simulink model "Woofer_Vented_L160_simscape"  (R2026a)
settings: Solver=ode23t  StopTime=0.2
libraries: fl_lib x21, nesl_utility x6
settings Model: Creator=mads  LastModifiedBy=mads
settings DataIOCC: ExternalInput=[(0:1e-4:0.2)' sin(2*pi*25*(0:1e-4:0.2)')]  LoadExternalInput=on

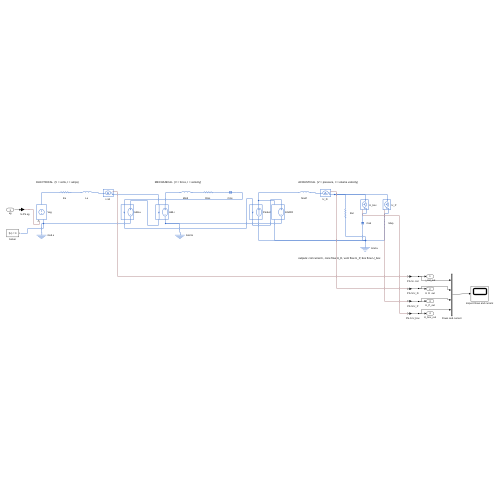
[thumbnail: Simulink's stored preview of the top-level diagram]
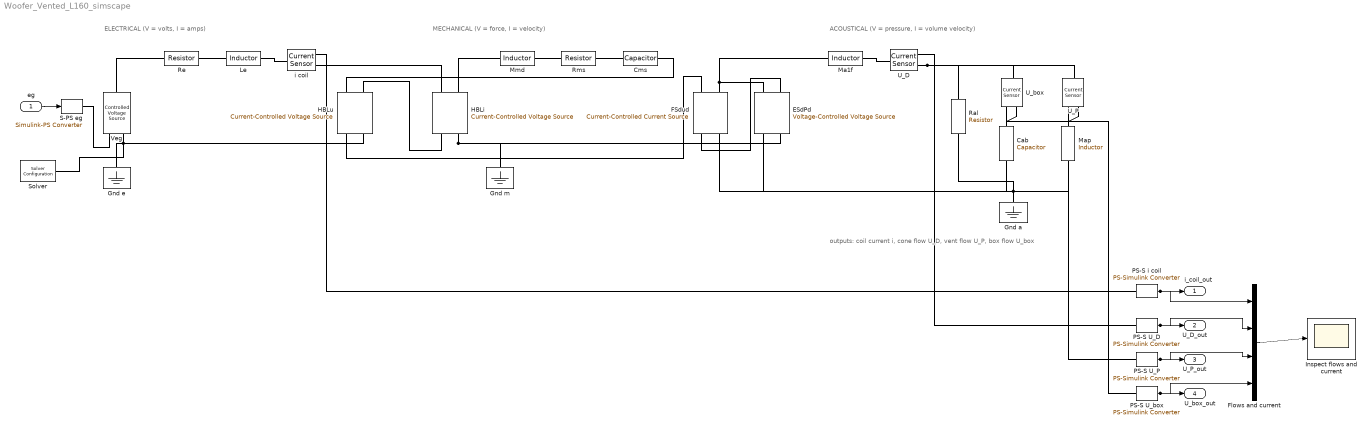
== system Woofer_Vented_L160_simscape ==
  note: ELECTRICAL (V = volts, I = amps)
  note: MECHANICAL (V = force, I = velocity)
  note: ACOUSTICAL (V = pressure, I = volume velocity)
  note: outputs: coil current i, cone flow U_D, vent flow U_P, box flow U_box
  eg : Inport
  Cab : fl_lib/Electrical/Electrical Elements/Capacitor  c=6.21e-07 F  r=0 Ohm  g=0 1/Ohm  i_specify=off  i_priority=None  i=0 A  i_nominal_specify=off  i_nominal_value=1  i_nominal_unit=A  v_specify=off  v_priority=None  v=0 V  v_nominal_specify=off  v_nominal_value=1  v_nominal_unit=V  vc_specify=off  vc_priority=High  vc=0 V  vc_nominal_specify=off  vc_nominal_value=1  vc_nominal_unit=V
  Cms : fl_lib/Electrical/Electrical Elements/Capacitor  c=0.0011735 F  r=0 Ohm  g=0 1/Ohm  i_specify=off  i_priority=None  i=0 A  i_nominal_specify=off  i_nominal_value=1  i_nominal_unit=A  v_specify=off  v_priority=None  v=0 V  v_nominal_specify=off  v_nominal_value=1  v_nominal_unit=V  vc_specify=off  vc_priority=High  vc=0 V  vc_nominal_specify=off  vc_nominal_value=1  vc_nominal_unit=V
  ESdPd : fl_lib/Electrical/Electrical Sources/Voltage-Controlled Voltage Source  K=0.034967  v1_specify=off  v1_priority=None  v1=0 V  v1_nominal_specify=off  v1_nominal_value=1  v1_nominal_unit=V  v2_specify=off  v2_priority=None  v2=0 V  v2_nominal_specify=off  v2_nominal_value=1  v2_nominal_unit=V
  FSdud : fl_lib/Electrical/Electrical Sources/Current-Controlled Current Source  K=0.034967  i1_specify=off  i1_priority=None  i1=0 A  i1_nominal_specify=off  i1_nominal_value=1  i1_nominal_unit=A  i2_specify=off  i2_priority=None  i2=0 A  i2_nominal_specify=off  i2_nominal_value=1  i2_nominal_unit=A
  Flows and current : Mux
  Gnd a : fl_lib/Electrical/Electrical Elements/Electrical Reference
  Gnd e : fl_lib/Electrical/Electrical Elements/Electrical Reference
  Gnd m : fl_lib/Electrical/Electrical Elements/Electrical Reference
  HBLi : fl_lib/Electrical/Electrical Sources/Current-Controlled Voltage Source  K=8.283 Ohm  i1_specify=off  i1_priority=None  i1=0 A  i1_nominal_specify=off  i1_nominal_value=1  i1_nominal_unit=A  v2_specify=off  v2_priority=None  v2=0 V  v2_nominal_specify=off  v2_nominal_value=1  v2_nominal_unit=V
  HBLu : fl_lib/Electrical/Electrical Sources/Current-Controlled Voltage Source  K=8.283 Ohm  i1_specify=off  i1_priority=None  i1=0 A  i1_nominal_specify=off  i1_nominal_value=1  i1_nominal_unit=A  v2_specify=off  v2_priority=None  v2=0 V  v2_nominal_specify=off  v2_nominal_value=1  v2_nominal_unit=V
  Inspect flows and current : Scope
  Le : fl_lib/Electrical/Electrical Elements/Inductor  l=0.001498 H  r=0 Ohm  g=0 1/Ohm  i_specify=off  i_priority=None  i=0 A  i_nominal_specify=off  i_nominal_value=1  i_nominal_unit=A  v_specify=off  v_priority=None  v=0 V  v_nominal_specify=off  v_nominal_value=1  v_nominal_unit=V  i_L_specify=off  i_L_priority=High  i_L=0 A  i_L_nominal_specify=off  i_L_nominal_value=1  i_L_nominal_unit=A
  Ma1f : fl_lib/Electrical/Electrical Elements/Inductor  l=3.084 H  r=0 Ohm  g=0 1/Ohm  i_specify=off  i_priority=None  i=0 A  i_nominal_specify=off  i_nominal_value=1  i_nominal_unit=A  v_specify=off  v_priority=None  v=0 V  v_nominal_specify=off  v_nominal_value=1  v_nominal_unit=V  i_L_specify=off  i_L_priority=High  i_L=0 A  i_L_nominal_specify=off  i_L_nominal_value=1  i_L_nominal_unit=A
  Map : fl_lib/Electrical/Electrical Elements/Inductor  l=67.44 H  r=348.9 Ohm  g=0 1/Ohm  i_specify=off  i_priority=None  i=0 A  i_nominal_specify=off  i_nominal_value=1  i_nominal_unit=A  v_specify=off  v_priority=None  v=0 V  v_nominal_specify=off  v_nominal_value=1  v_nominal_unit=V  i_L_specify=off  i_L_priority=High  i_L=0 A  i_L_nominal_specify=off  i_L_nominal_value=1  i_L_nominal_unit=A
  Mmd : fl_lib/Electrical/Electrical Elements/Inductor  l=0.03668 H  r=0 Ohm  g=0 1/Ohm  i_specify=off  i_priority=None  i=0 A  i_nominal_specify=off  i_nominal_value=1  i_nominal_unit=A  v_specify=off  v_priority=None  v=0 V  v_nominal_specify=off  v_nominal_value=1  v_nominal_unit=V  i_L_specify=off  i_L_priority=High  i_L=0 A  i_L_nominal_specify=off  i_L_nominal_value=1  i_L_nominal_unit=A
  PS-S U_D : nesl_utility/PS-Simulink Converter  PhysicalDomain=network_engine_domain  SubClassName=ps_output  LeftPortType=input  RightPortType=output  PseudoPeriodic=off  Frequencies=[]  VectorFormat=inherit  Unit=A  AffineConversion=off
  PS-S U_P : nesl_utility/PS-Simulink Converter  PhysicalDomain=network_engine_domain  SubClassName=ps_output  LeftPortType=input  RightPortType=output  PseudoPeriodic=off  Frequencies=[]  VectorFormat=inherit  Unit=A  AffineConversion=off
  PS-S U_box : nesl_utility/PS-Simulink Converter  PhysicalDomain=network_engine_domain  SubClassName=ps_output  LeftPortType=input  RightPortType=output  PseudoPeriodic=off  Frequencies=[]  VectorFormat=inherit  Unit=A  AffineConversion=off
  PS-S i coil : nesl_utility/PS-Simulink Converter  PhysicalDomain=network_engine_domain  SubClassName=ps_output  LeftPortType=input  RightPortType=output  PseudoPeriodic=off  Frequencies=[]  VectorFormat=inherit  Unit=A  AffineConversion=off
  Ral : fl_lib/Electrical/Electrical Elements/Resistor  R=66114 Ohm  i_specify=off  i_priority=None  i=0 A  i_nominal_specify=off  i_nominal_value=1  i_nominal_unit=A  v_specify=off  v_priority=None  v=0 V  v_nominal_specify=off  v_nominal_value=1  v_nominal_unit=V
  Re : fl_lib/Electrical/Electrical Elements/Resistor  R=5.7 Ohm  i_specify=off  i_priority=None  i=0 A  i_nominal_specify=off  i_nominal_value=1  i_nominal_unit=A  v_specify=off  v_priority=None  v=0 V  v_nominal_specify=off  v_nominal_value=1  v_nominal_unit=V
  Rms : fl_lib/Electrical/Electrical Elements/Resistor  R=0.6085 Ohm  i_specify=off  i_priority=None  i=0 A  i_nominal_specify=off  i_nominal_value=1  i_nominal_unit=A  v_specify=off  v_priority=None  v=0 V  v_nominal_specify=off  v_nominal_value=1  v_nominal_unit=V
  S-PS eg : nesl_utility/Simulink-PS Converter  PhysicalDomain=network_engine_domain  SubClassName=ps_input  LeftPortType=input  RightPortType=output  PseudoPeriodic=off  Frequencies=[]  NoiseDistribution=none  NoiseParameters=[]  Unit=V  AffineConversion=off  FilteringAndDerivatives=provide  SimscapeFilterOrder=1  InputFilterTimeConstant=0.001  UdotUserProvided=0
  Solver : nesl_utility/Solver Configuration  PhysicalDomain=network_engine_domain  SubClassName=solver  LeftPortType=input  RightPortType=generic  Tones=[]  Harmonics=[]  SimulateNoise=off  Profile=off  UseLocalSampling=off  EnableSwitchedLinearOptims=on  FrequencyDomain=off  UseCCode=off  RelTol=0.001  AbsTol=0.001  MinStep=1e-09  ToWorkspace=off  RevertToSquareIcSolve=off  NumHomotopyIterations=100  PhasorMode=off  PhasorModeNumHarmonics=1  ConsistencySolver=NEWTON_XTOL_AFTER_FTOL  CanonicalOrdering=CANONICAL  OptimizeIntermediates=OPTIMIZED  IndexReductionMethod=DerivativeReplacement  DoDC=off  ResidualTolerance=1e-09  ConsistencyTolSource=GLOBAL  ConsistencyAbsTol=0.001  ConsistencyRelTol=0.001  ConsistencyTolFactor=0.001  UseLocalSolver=off  LocalSolverChoice=NE_BACKWARD_EULER_ADVANCER  ResolveIndetEquations=on  FunctionEvalNumThread=1  LocalSolverSampleTime=0.001  DoFixedCost=off  MaxNonlinIter=3  MaxModeIter=2  ComputeImpulses=off  ImpulseIterations=2  LinearAlgebra=auto  LinearAlgebraNumThread=0  EquationFormulation=NE_TIME_EF  DelaysMemoryBudget=1024  AutomaticFiltering=on  FilteringTimeConstant=0.001  PartitionStorageMethod=AS_NEEDED  PartitionMemoryBudget=1024  PartitionMethod=ROBUST  MultibodyUseLocalSolver=off  MultibodyLocalSolverChoice=ODE1  MultibodyLocalSolverSampleTime=0.001
  U_D : fl_lib/Electrical/Electrical Sensors/Current Sensor
  U_P : fl_lib/Electrical/Electrical Sensors/Current Sensor
  U_box : fl_lib/Electrical/Electrical Sensors/Current Sensor
  Veg : fl_lib/Electrical/Electrical Sources/Controlled Voltage Source
  i coil : fl_lib/Electrical/Electrical Sensors/Current Sensor
  i_coil_out : Outport
  U_D_out : Outport  Port=2
  U_P_out : Outport  Port=3
  U_box_out : Outport  Port=4
  wires:
  eg/1 -> S-PS eg/1
  PS-S i coil/1 -> i_coil_out/1, Flows and current/1
  PS-S U_D/1 -> U_D_out/1, Flows and current/2
  PS-S U_P/1 -> U_P_out/1, Flows and current/3
  PS-S U_box/1 -> U_box_out/1, Flows and current/4
  Flows and current/1 -> Inspect flows and current/1
  connections:
  S-PS eg/RConn1 -- Veg/RConn1
  Veg/LConn1 -- Re/LConn1
  Re/RConn1 -- Le/LConn1
  Le/RConn1 -- i coil/LConn1
  i coil/RConn2 -- HBLi/LConn1
  HBLi/RConn1 -- HBLu/LConn2
  HBLu/RConn2 -- Gnd e/LConn1 -- Veg/RConn2 -- Solver/RConn1
  HBLi/LConn2 -- Mmd/LConn1
  Mmd/RConn1 -- Rms/LConn1
  Rms/RConn1 -- Cms/LConn1
  Cms/RConn1 -- HBLu/LConn1
  HBLu/RConn1 -- FSdud/LConn1
  FSdud/RConn1 -- ESdPd/LConn2
  HBLi/RConn2 -- ESdPd/RConn2 -- Gnd m/LConn1
  Ma1f/LConn1 -- FSdud/LConn2 -- ESdPd/LConn1
  Ma1f/RConn1 -- U_D/LConn1
  Ral/LConn1 -- U_D/RConn2 -- U_box/LConn1 -- U_P/LConn1
  Ral/RConn1 -- Cab/RConn1 -- Map/RConn1 -- FSdud/RConn2 -- Gnd a/LConn1 -- ESdPd/RConn1
  U_box/RConn2 -- Cab/LConn1
  U_P/RConn2 -- Map/LConn1
  i coil/RConn1 -- PS-S i coil/LConn1
  U_D/RConn1 -- PS-S U_D/LConn1
  U_P/RConn1 -- PS-S U_P/LConn1
  U_box/RConn1 -- PS-S U_box/LConn1
